simulink model "untitled1"  (R2024b)
settings: Solver=VariableStepAuto  StartTime=0.0  StopTime=0.06  RelTol=1e-3
libraries: spsVoltageMeasurementLib x2, spsACVoltageSourceLib x1, spsCurrentMeasurementLib x1, spsSeriesRLCBranchLib x1, spsThyristorLib x1, sps_lib x1
settings Model: Creator=SURAJ KUMAR  LastModifiedBy=SURAJ KUMAR

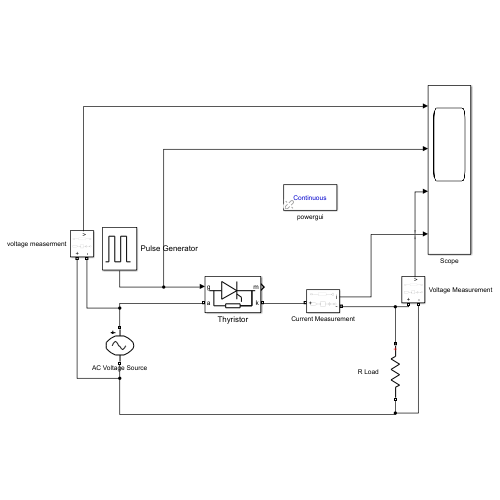
[thumbnail: Simulink's stored preview of the top-level diagram]
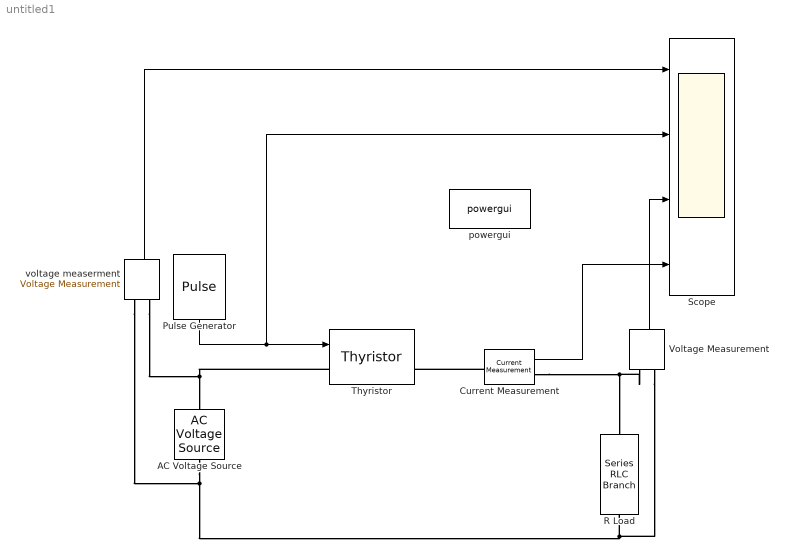
== system untitled1 ==
  AC Voltage Source : spsACVoltageSourceLib/AC Voltage Source  Amplitude=120*sqrt(2)  Phase=0  Frequency=60  SampleTime=0  Measurements=None  BusType=swing  Pref=10e3  Qref=0  Qmin=-inf  Qmax=+inf
  Current Measurement : spsCurrentMeasurementLib/Current Measurement  PhasorSimulation=off  OutputType=Complex  PSBequivalent=0
  Pulse Generator : DiscretePulseGenerator  PulseType=Time based  Period=0.0166  PulseWidth=5  PhaseDelay=0.0028
  R Load : spsSeriesRLCBranchLib/Series RLC Branch  LConnTagsString=__new0  RConnTagsString=__new0  BranchType=R  Resistance=100  Inductance=1e-3  SetiL0=off  InitialCurrent=0  Capacitance=1e-6  Setx0=off  InitialVoltage=0  Measurements=None
  Scope : Scope  NumInputPorts=4
  Thyristor : spsThyristorLib/Thyristor  Ron=0.001  Lon=0  Vf=0.8  IC=0  Rs=500  Cs=250e-9  Measurements=on
  Voltage Measurement : spsVoltageMeasurementLib/Voltage Measurement  PhasorSimulation=off  OutputType=Complex  PSBequivalent=0
  powergui : sps_lib/powergui  Priority=1  SimulationMode=Continuous  SampleTime=50e-6  frequency=60  Iterations=50  frequencyindice=60  Pbase=100e6  ErrMax=1e-4  UnitsV=kV  UnitsW=MW  buscounter=0  FunctionMessages=off  echomessages=off  EnableUseOfTLC=off  CurrentSourceSwitches=off  DisableSnubberDevices=off  DisableRonSwitches=off  DisableVfSwitches=off  DisplayEquations=off  AutomaticDiscreteSolvers=off  SolverType=Tustin/Backward Euler (TBE)  Interpol=off  ExternalGateDelay=off  methode=off  Ts=100  x0status=blocks  SPID=on  SwTol=0  HookPort=off  NonlinearTolerance=1e-4  nMaxIteration=100  ContinueOnMaxIteration=off  RestoreLinks=warning  ResistiveCurrentMeasurement=off  Frange=[0:2:500]  Ylog=off  Xlog=on  ShowGrid=off  save=off  variable=ZData  structure=0  ZoomFFT=off  StartTime=0.0  cycles=1  DisplayStyle=1  fundamental=60  FreqAxis=off  MaxFrequency=1000  frequencyindicesteady=1  RmsSteady=1  display=off
  voltage measerment : spsVoltageMeasurementLib/Voltage Measurement  PhasorSimulation=off  OutputType=Complex  PSBequivalent=0
  wires:
  Pulse Generator/1 -> Thyristor/1, Scope/2
  voltage measerment/1 -> Scope/1
  Voltage Measurement/1 -> Scope/3
  Current Measurement/1 -> Scope/4
  connections:
  Thyristor/LConn1 -- AC Voltage Source/RConn1 -- voltage measerment/LConn2
  AC Voltage Source/LConn1 -- Voltage Measurement/LConn2 -- R Load/RConn1 -- voltage measerment/LConn1
  Current Measurement/LConn1 -- Thyristor/RConn1
  Current Measurement/RConn1 -- R Load/LConn1 -- Voltage Measurement/LConn1
